simulink model "nms_sim_2D_cost"  (R2024b)
settings: Solver=ode15s  StartTime=0.0  StopTime=t_sim  MaxStep=dt_max  EnableMultiTasking=on
values from neighbouring files (symbols this model uses):
  a_BFSH = param_ctrl(35)*1    [setCtrlPar_optim_CPGreflex2001_2D.m]
  a_GAS = param_ctrl(37)*1    [setCtrlPar_optim_CPGreflex2001_2D.m]
  a_GLU = param_ctrl(31)*1    [setCtrlPar_optim_CPGreflex2001_2D.m]
  a_HAM = param_ctrl(33)*1    [setCtrlPar_optim_CPGreflex2001_2D.m]
  a_HFL = param_ctrl(32)*1    [setCtrlPar_optim_CPGreflex2001_2D.m]
  a_RF = param_ctrl(34)*1    [setCtrlPar_optim_CPGreflex2001_2D.m]
  a_SOL = param_ctrl(38)*1    [setCtrlPar_optim_CPGreflex2001_2D.m]
  a_TA = param_ctrl(39)*1    [setCtrlPar_optim_CPGreflex2001_2D.m]
  a_VAS = param_ctrl(36)*1    [setCtrlPar_optim_CPGreflex2001_2D.m]
  ai = param_ctrl(96)*2.0    [setCtrlPar_optim_CPGreflex2001_2D.m]
  b_BFSH = param_ctrl(52)*.51    [setCtrlPar_optim_CPGreflex2001_2D.m]
  b_BFSHGAS = param_ctrl(55)*.51    [setCtrlPar_optim_CPGreflex2001_2D.m]
  b_BFSHHAM = param_ctrl(54)*.51    [setCtrlPar_optim_CPGreflex2001_2D.m]
  b_BFSHVAS = param_ctrl(53)*.51    [setCtrlPar_optim_CPGreflex2001_2D.m]
  b_GAS = param_ctrl(59)*.51    [setCtrlPar_optim_CPGreflex2001_2D.m]
  b_GASBFSH = param_ctrl(60)*.51    [setCtrlPar_optim_CPGreflex2001_2D.m]
  b_GASSOL = param_ctrl(61)*.51    [setCtrlPar_optim_CPGreflex2001_2D.m]
  b_GLU = param_ctrl(40)*.51    [setCtrlPar_optim_CPGreflex2001_2D.m]
  b_GLUHAM = param_ctrl(42)*.51    [setCtrlPar_optim_CPGreflex2001_2D.m]
  b_GLUHFL = param_ctrl(41)*.51    [setCtrlPar_optim_CPGreflex2001_2D.m]
  b_HAM = param_ctrl(46)*.51    [setCtrlPar_optim_CPGreflex2001_2D.m]
  b_HAMBFSH = param_ctrl(48)*.51    [setCtrlPar_optim_CPGreflex2001_2D.m]
  b_HAMGLU = param_ctrl(47)*.51    [setCtrlPar_optim_CPGreflex2001_2D.m]
  b_HFL = param_ctrl(43)*.51    [setCtrlPar_optim_CPGreflex2001_2D.m]
  b_HFLGLU = param_ctrl(44)*.51    [setCtrlPar_optim_CPGreflex2001_2D.m]
  b_HFLRF = param_ctrl(45)*.51    [setCtrlPar_optim_CPGreflex2001_2D.m]
  b_RF = param_ctrl(49)*.51    [setCtrlPar_optim_CPGreflex2001_2D.m]
  b_RFHFL = param_ctrl(50)*.51    [setCtrlPar_optim_CPGreflex2001_2D.m]
  b_RFVAS = param_ctrl(51)*.51    [setCtrlPar_optim_CPGreflex2001_2D.m]
  b_SOL = param_ctrl(62)*.51    [setCtrlPar_optim_CPGreflex2001_2D.m]
  b_SOLGAS = param_ctrl(64)*.51    [setCtrlPar_optim_CPGreflex2001_2D.m]
  b_SOLTA = param_ctrl(63)*.51    [setCtrlPar_optim_CPGreflex2001_2D.m]
  b_TA = param_ctrl(65)*.51    [setCtrlPar_optim_CPGreflex2001_2D.m]
  b_TASOL = param_ctrl(66)*.51    [setCtrlPar_optim_CPGreflex2001_2D.m]
  b_VAS = param_ctrl(56)*.51    [setCtrlPar_optim_CPGreflex2001_2D.m]
  b_VASBFSH = param_ctrl(57)*.51    [setCtrlPar_optim_CPGreflex2001_2D.m]
  b_VASRF = param_ctrl(58)*.51    [setCtrlPar_optim_CPGreflex2001_2D.m]
  bias = param_ctrl(97)*2.5    [setCtrlPar_optim_CPGreflex2001_2D.m]
  c = 0.05    [nms_MS_2D_scaled.m]
  c_jointstop = 0.3 / (pi/180)    (= 17.1887338539)    [nms_MS_2D_scaled.m]
  D12_F = 0.16    *scaleL_JPhys    [nms_MechInit_2D_scaleSkel.m]
  D12_S = 0.2460	*sub_height    [nms_MechInit_2D_scaleSkel.m]
  D12_T = 0.2450  *sub_height    [nms_MechInit_2D_scaleSkel.m]
  D12y_F = 0.039  *sub_height    [nms_MechInit_2D_scaleSkel.m]
  D12z_HAT = 0.1    [nms_MS_2D_scaled.m]
  D13_F = 0.20    *scaleL_JPhys    [nms_MechInit_2D_scaleSkel.m]
  D1G_F = 0.14    *scaleL_JPhys    [nms_MechInit_2D_scaleSkel.m]
  D1G_HAT = 0.35  *scaleL_JPhys    [nms_MechInit_2D_scaleSkel.m]
  D1G_S = (0.3 - D12y_F/4)	*scaleL_JPhys    [nms_MechInit_2D_scaleSkel.m]
  D1G_T = (0.3 - D12y_F/4)	*scaleL_JPhys    [nms_MechInit_2D_scaleSkel.m]
  D1Gy_F = D12y_F*D1G_F/D12_F    (= 0.07)    [nms_MechInit_2D_scaleSkel.m]
  d_BFSH = param_ctrl(26)*1    [setCtrlPar_optim_CPGreflex2001_2D.m]
  d_GAS = param_ctrl(28)*1    [setCtrlPar_optim_CPGreflex2001_2D.m]
  d_GLU = param_ctrl(22)*1    [setCtrlPar_optim_CPGreflex2001_2D.m]
  d_HAM = param_ctrl(24)*1    [setCtrlPar_optim_CPGreflex2001_2D.m]
  d_HFL = param_ctrl(23)*1    [setCtrlPar_optim_CPGreflex2001_2D.m]
  d_RF = param_ctrl(25)*1    [setCtrlPar_optim_CPGreflex2001_2D.m]
  d_SOL = param_ctrl(29)*1    [setCtrlPar_optim_CPGreflex2001_2D.m]
  d_TA = param_ctrl(30)*1    [setCtrlPar_optim_CPGreflex2001_2D.m]
  d_VAS = param_ctrl(27)*1    [setCtrlPar_optim_CPGreflex2001_2D.m]
  DeltaThRef = 5e-3    (= 0.005)    [nms_MS_2D_scaled.m]
  dloptBFSH = 3.0    (= 3)    [setCtrlPar_optim_CPGreflex2001_2D.m]
  dloptGAS = 3.0    (= 3)    [setCtrlPar_optim_CPGreflex2001_2D.m]
  dloptGLU = 3.0    (= 3)    [setCtrlPar_optim_CPGreflex2001_2D.m]
  dloptHAM = 3.0    (= 3)    [setCtrlPar_optim_CPGreflex2001_2D.m]
  dloptHFL = 3.0    (= 3)    [setCtrlPar_optim_CPGreflex2001_2D.m]
  dloptRF = 3.0    (= 3)    [setCtrlPar_optim_CPGreflex2001_2D.m]
  dloptSOL = 3.0    (= 3)    [setCtrlPar_optim_CPGreflex2001_2D.m]
  dloptTA = 3.0    (= 3)    [setCtrlPar_optim_CPGreflex2001_2D.m]
  dloptVAS = 3.0    (= 3)    [setCtrlPar_optim_CPGreflex2001_2D.m]
  ec_BFSH = param_ctrl(80)*0.15    [setCtrlPar_optim_CPGreflex2001_2D.m]
  ec_GAS = param_ctrl(82)*0.15    [setCtrlPar_optim_CPGreflex2001_2D.m]
  ec_GLU = param_ctrl(76)*0.15    [setCtrlPar_optim_CPGreflex2001_2D.m]
  ec_HAM = param_ctrl(78)*0.15    [setCtrlPar_optim_CPGreflex2001_2D.m]
  ec_HFL = param_ctrl(77)*0.15    [setCtrlPar_optim_CPGreflex2001_2D.m]
  ec_RF = param_ctrl(79)*0.15    [setCtrlPar_optim_CPGreflex2001_2D.m]
  ec_TA = param_ctrl(84)*0.15    [setCtrlPar_optim_CPGreflex2001_2D.m]
  ec_VAS = param_ctrl(81)*0.15    [setCtrlPar_optim_CPGreflex2001_2D.m]
  eref = 0.04    [nms_MS_2D_scaled.m]
  eref_GAS = 0.1    [nms_MS_2D_scaled.m]
  eref_SOL = 0.1    [nms_MS_2D_scaled.m]
  es_BFSH = param_ctrl(89)*0.15    [setCtrlPar_optim_CPGreflex2001_2D.m]
  es_GAS = param_ctrl(91)*0.15    [setCtrlPar_optim_CPGreflex2001_2D.m]
  es_GLU = param_ctrl(85)*0.15    [setCtrlPar_optim_CPGreflex2001_2D.m]
  es_HAM = param_ctrl(87)*0.15    [setCtrlPar_optim_CPGreflex2001_2D.m]
  es_HFL = param_ctrl(86)*0.15    [setCtrlPar_optim_CPGreflex2001_2D.m]
  es_RF = param_ctrl(88)*0.15    [setCtrlPar_optim_CPGreflex2001_2D.m]
  es_TA = param_ctrl(93)*0.15    [setCtrlPar_optim_CPGreflex2001_2D.m]
  es_VAS = param_ctrl(90)*0.15    [setCtrlPar_optim_CPGreflex2001_2D.m]
  FmaxBFSH = 350    [nms_MS_2D_scaled.m]
  FmaxGAS = 2000    [nms_MS_2D_scaled.m]
  FmaxGLU = 4000    [nms_MS_2D_scaled.m]
  FmaxHAM = 2000    [nms_MS_2D_scaled.m]
  FmaxHFL = 2000    [nms_MS_2D_scaled.m]
  FmaxRF = 850    [nms_MS_2D_scaled.m]
  FmaxSOL = 4000    [nms_MS_2D_scaled.m]
  FmaxTA = 800    [nms_MS_2D_scaled.m]
  FmaxVAS = 5000    [nms_MS_2D_scaled.m]
  g = 9.81    [nms_MS_2D_scaled.m]
  gamma_4 = param_ctrl(11) * 1.7    [setCtrlPar_optim_CPGreflexsynergy2023_2D.m]
  h_BFSH = param_ctrl(71)*.1    [setCtrlPar_optim_CPGreflex2001_2D.m]
  h_GAS = param_ctrl(73)*.1    [setCtrlPar_optim_CPGreflex2001_2D.m]
  h_GLU = param_ctrl(67)*.1    [setCtrlPar_optim_CPGreflex2001_2D.m]
  h_HAM = param_ctrl(69)*.1    [setCtrlPar_optim_CPGreflex2001_2D.m]
  h_HFL = param_ctrl(68)*.1    [setCtrlPar_optim_CPGreflex2001_2D.m]
  h_RF = param_ctrl(70)*.1    [setCtrlPar_optim_CPGreflex2001_2D.m]
  h_SOL = param_ctrl(74)*.1    [setCtrlPar_optim_CPGreflex2001_2D.m]
  h_TA = param_ctrl(75)*.1    [setCtrlPar_optim_CPGreflex2001_2D.m]
  h_VAS = param_ctrl(72)*.1    [setCtrlPar_optim_CPGreflex2001_2D.m]
  HLCtrlPar = [theta_tgt l_clr alpha_tgt alpha_cd alpha_cv]    [setCtrlPar_optim_reflex2015_2D.m]
  In_F = 0.005    *scaleM*scaleL_JPhys^2    [nms_MechInit_2D_scaleSkel.m]
  In_HAT = 2.5    *scaleM*scaleL_JPhys^2    [nms_MechInit_2D_scaleSkel.m]
  In_S = 0.05     *scaleM*scaleL_JPhys^2    [nms_MechInit_2D_scaleSkel.m]
  In_T = 0.15     *scaleM*scaleL_JPhys^2    [nms_MechInit_2D_scaleSkel.m]
  init_exc = 0.01    [setInitPar_optim_2D.m]
  init_fm = 0.01    [setInitPar_optim_2D.m]
  init_lce = 1    [setInitPar_optim_2D.m]
  init_LCPG = param_ctrl(12) * 0.01    [setCtrlPar_optim_CPGreflexsynergy2023_2D.m]
  init_LStance = 1    [setInitPar_optim_2D.m]
  init_N1 = osc_signal1(phi_off_osc_ind)    [setCtrlPar_optim_CPGreflex2001_2D.m]
  ... (+441 more)
undefined symbols (not defined in the file or in its folder): cost_act_exponent, cost_v_tgt, flag_controller, Newton, nStep_obj, nStep_startKin, Raphson, sgn, SSW_kin, terrain_slope_angle, v_plateS1, X, Y, Z
libraries: nesl_utility x94, sm_lib x90, simulink x28, simulink_extras x12
(part 19 of 20)

== system nms_sim_2D_cost/Reflex Controller/Lower Control Layer (Spinal Cord)/R Swing Phase ==
  note: Left Swing Phase Control
  note: 0: Pre-excitations
  note: M6: swing hip
  note: M7: flex knee
  note: M8: hold knee
  note: M9: stop leg
  note: M10: prepare stance
  note: M5: flex ankle
  CtrlPar : Inport
  Stance : Inport  Port=2
  a_tgt : Inport  Port=3
  l_clr : Inport  Port=4
  LceRF : Inport  Port=5
  VceRF : Inport  Port=6
  LceHAM : Inport  Port=7
  VceHAM : Inport  Port=8
  lceBFSH : Inport  Port=9
  VceVAS : Inport  Port=10
  VceBFSH : Inport  Port=11
  LceHFL : Inport  Port=12
  LceGLU : Inport  Port=13
  LceVAS : Inport  Port=14
  LceTA : Inport  Port=15
  Enable : EnablePort  StatesWhenEnabling=reset  ZeroCross=off
  Constant1 : Constant  Value=0  OutDataTypeStr=boolean
  Constant10 : Constant  Value=leg_l
  Constant2 : Constant
  Constant3 : Constant
  Constant5 : Constant
  Demux1 : Demux  Outputs=2
  Demux2 : Demux  Outputs=2
  Demux4 : Demux  Outputs=9
  Divide{1..8,22} (9 alike) : Product
  Gain1 : Gain  Gain=-1
  Logical Operator : Logic  Operator=NOT  AllPortsSameDT=off  OutDataTypeStr=boolean
  Logical Operator1 : Logic  AllPortsSameDT=off  OutDataTypeStr=boolean
  Logical Operator2 : Logic  Operator=NOT  AllPortsSameDT=off  OutDataTypeStr=boolean
  Mux1 : Mux  Inputs=3
  Mux2 : Mux  Inputs=2
  Mux3 : Mux  Inputs=2
  Mux4 : Mux  Inputs=3
  Mux8 : Mux  Inputs=2
  Relational Operator : RelationalOperator  Operator=<=  OutDataTypeStr=boolean  ZeroCross=off  InputSameDT=off
  S-R Flip-Flop : simulink_extras/Flip Flops/S-R Flip-Flop  initial_condition=0
  Sum1 : Sum  Inputs=-+|  InputSameDT=on  SaturateOnIntegerOverflow=on  OutDataTypeStr=Inherit: Same as first input
  Sum10 : Sum  Inputs=++|  InputSameDT=on  SaturateOnIntegerOverflow=on  OutDataTypeStr=Inherit: Same as first input
  Sum13 : Sum  Inputs=|+-  InputSameDT=on  SaturateOnIntegerOverflow=on  OutDataTypeStr=Inherit: Same as first input
  Sum14 : Sum  Inputs=|+-  InputSameDT=on  SaturateOnIntegerOverflow=on  OutDataTypeStr=Inherit: Same as first input
  Sum2 : Sum  Inputs=++|  InputSameDT=on  SaturateOnIntegerOverflow=on  OutDataTypeStr=Inherit: Same as first input
  Sum3 : Sum  Inputs=-+|  InputSameDT=on  SaturateOnIntegerOverflow=on  OutDataTypeStr=Inherit: Same as first input
  Sum4 : Sum  Inputs=|+-  InputSameDT=on  SaturateOnIntegerOverflow=on  OutDataTypeStr=Inherit: Same as first input
  Sum5 : Sum  Inputs=+-|  InputSameDT=on  SaturateOnIntegerOverflow=on  OutDataTypeStr=Inherit: Same as first input
  Sum6 : Sum  Inputs=|++  InputSameDT=on  SaturateOnIntegerOverflow=on  OutDataTypeStr=Inherit: Same as first input
  Sum7 : Sum  Inputs=|++  InputSameDT=on  SaturateOnIntegerOverflow=on  OutDataTypeStr=Inherit: Same as first input
  Sum8 : Sum  Inputs=++|  InputSameDT=on  SaturateOnIntegerOverflow=on  OutDataTypeStr=Inherit: Same as first input
  Sum9 : Sum  Inputs=+-|  InputSameDT=on  SaturateOnIntegerOverflow=on  OutDataTypeStr=Inherit: Same as first input
  Terminator : Terminator
  kneei_flexion from alpha : Subsystem  TreatAsAtomicUnit=on
  kneeii_damp and hold & kneeiii_leg stop & kneeiv_stance preparation : Subsystem  TreatAsAtomicUnit=on
  negative half : Saturate  UpperLimit=0  LowerLimit=-inf  ZeroCross=off
  negative half1 : Saturate  UpperLimit=0  LowerLimit=-inf  ZeroCross=off
  negative half2 : Saturate  UpperLimit=0  LowerLimit=-inf  ZeroCross=off
  parSwA : Selector  InputPortWidth=Sw_i  IndexOptions=Index vector (dialog)  Indices=parSwA_i  OutputSizes=1
  parSwH : Selector  InputPortWidth=Sw_i  IndexOptions=Index vector (dialog)  Indices=parSwH_i  OutputSizes=1
  parSwKi : Selector  InputPortWidth=Sw_i  IndexOptions=Index vector (dialog)  Indices=parSwKi_i  OutputSizes=1
  parSwPhi : Selector  InputPortWidth=Sw_i  IndexOptions=Index vector (dialog)  Indices=parSwPhi_i  OutputSizes=1
  parSwPreE : Selector  InputPortWidth=Sw_i  IndexOptions=Index vector (dialog)  Indices=parSwPreE_i  OutputSizes=1
  phi_clr : Fcn  Expr=acos((u(2)^2+u(3)^2-u(1)^2)/(2*u(2)*u(3)))
  positive half1 : Saturate  UpperLimit=inf  LowerLimit=0  ZeroCross=off
  positive half2 : Saturate  UpperLimit=inf  LowerLimit=0  ZeroCross=off
  positive half3 : Saturate  UpperLimit=inf  LowerLimit=0  ZeroCross=off
  E_Sw_0 : Outport  OutputWhenDisabled=reset  InitialOutput=0  VectorParamsAs1DForOutWhenUnconnected=off
  E_M5_Sw [TA] : Outport  Port=2  OutputWhenDisabled=reset  InitialOutput=0  VectorParamsAs1DForOutWhenUnconnected=off
  E_M6 [HFL GLU] : Outport  Port=3  OutputWhenDisabled=reset  InitialOutput=0  VectorParamsAs1DForOutWhenUnconnected=off
  E_M7_DS [BFSH] : Outport  Port=4  OutputWhenDisabled=reset  InitialOutput=0  VectorParamsAs1DForOutWhenUnconnected=off
  E_M7_Sw [BFSH] : Outport  Port=5  OutputWhenDisabled=reset  InitialOutput=0  VectorParamsAs1DForOutWhenUnconnected=off
  M8 [RF BFSH] : Outport  Port=6  OutputWhenDisabled=reset  InitialOutput=0  VectorParamsAs1DForOutWhenUnconnected=off
  M9 [HAM BFSH GAS] : Outport  Port=7  OutputWhenDisabled=reset  InitialOutput=0  VectorParamsAs1DForOutWhenUnconnected=off
  M10 [HFL GLU VAS] : Outport  Port=8  OutputWhenDisabled=reset  InitialOutput=0  VectorParamsAs1DForOutWhenUnconnected=off
  wires:
  CtrlPar/1 -> parSwA/1, parSwPreE/1, parSwH/1, kneeii_damp and hold & kneeiii_leg stop & kneeiv_stance preparation/1(CtrlPar), parSwPhi/1, parSwKi/1
  parSwH/1 -> Demux4/1
  Constant5/1 -> Sum10/1
  a_tgt/1 -> Sum2/1, kneeii_damp and hold & kneeiii_leg stop & kneeiv_stance preparation/2(a_tgt), Sum13/1
  Demux4/2 -> Sum13/2  "aRef_RF"
  Sum13/1 -> Divide22/2
  Demux4/1 -> Divide22/1  "a2lopt_RF"
  Divide22/1 -> Sum10/2
  Sum10/1 -> Sum1/1  "lceOffRF"
  Sum1/1 -> positive half2/1  "del_LceRF"
  positive half2/1 -> Divide5/1  "del_lce"
  Demux4/3 -> Divide5/2  "LGainRF_HFL"
  Demux4/6 -> Sum2/2  "a_del"
  Sum2/1 -> Sum4/1  "a_thr"
  Demux4/7 -> Sum4/2  "aRef_HAM"
  Sum4/1 -> Divide1/2
  Demux4/5 -> Divide1/1  "a2lopt_HAM"
  Constant2/1 -> Sum5/1
  Divide1/1 -> Sum5/2
  Sum3/1 -> positive half1/1
  positive half1/1 -> Divide2/1
  Demux4/8 -> Divide2/2  "LGainHAM_GLU"
  Sum5/1 -> Sum3/1  "lceOffHAM"
  LceHAM/1 -> Sum3/2, kneeii_damp and hold & kneeiii_leg stop & kneeiv_stance preparation/4(LceHAM)
  Gain1/1 -> Divide3/1
  negative half/1 -> Gain1/1  "-VceRF"
  parSwKi/1 -> Divide3/2  "VGainRF_BFSH"
  Divide3/1 -> kneei_flexion from alpha/1(SBFSH), E_M7_DS [BFSH]/1  "BFSH"
  Constant1/1 -> S-R Flip-Flop/2
  S-R Flip-Flop/2 -> Terminator/1
  S-R Flip-Flop/1 -> Logical Operator/1, kneeii_damp and hold & kneeiii_leg stop & kneeiv_stance preparation/Enable
  Logical Operator/1 -> kneei_flexion from alpha/Enable
  lceBFSH/1 -> Relational Operator/1
  Mux8/1 -> phi_clr/1
  l_clr/1 -> Mux8/1
  Constant10/1 -> Mux8/2
  parSwPhi/1 -> Demux1/1
  Sum9/1 -> Divide4/2
  Demux1/1 -> Divide4/1  "phi2lopt_BFSH"
  Demux1/2 -> Sum9/2  "phiRef_BFSH"
  phi_clr/1 -> Sum9/1
  Constant3/1 -> Sum8/1
  Divide4/1 -> Sum8/2
  Sum8/1 -> Relational Operator/2  "lceOffLClr_BFSH"
  VceBFSH/1 -> kneeii_damp and hold & kneeiii_leg stop & kneeiv_stance preparation/7(VceBFSH)
  LceHFL/1 -> kneeii_damp and hold & kneeiii_leg stop & kneeiv_stance preparation/9(LceHFL)  "LceHFL"
  LceGLU/1 -> kneeii_damp and hold & kneeiii_leg stop & kneeiv_stance preparation/10(LceGLU)
  LceVAS/1 -> kneeii_damp and hold & kneeiii_leg stop & kneeiv_stance preparation/11(LceVAS)
  kneeii_damp and hold & kneeiii_leg stop & kneeiv_stance preparation/6(SHFL_Sw_kiv) -> Mux1/1
  kneeii_damp and hold & kneeiii_leg stop & kneeiv_stance preparation/7(SGLU_Sw_kiv) -> Mux1/2
  kneei_flexion from alpha/1(SBFSH_Sw_ki) -> E_M7_Sw [BFSH]/1
  kneeii_damp and hold & kneeiii_leg stop & kneeiv_stance preparation/2(SBFSH_Sw_kii) -> Mux3/2
  kneeii_damp and hold & kneeiii_leg stop & kneeiv_stance preparation/4(SBFSH_Sw_kiii) -> Mux4/2
  parSwA/1 -> Demux2/1
  Demux2/1 -> Divide6/1  "LGainTA"
  Sum14/1 -> positive half3/1
  LceTA/1 -> Sum14/1
  positive half3/1 -> Divide6/2
  Demux2/2 -> Sum14/2  "LceOffTA"
  Logical Operator1/1 -> S-R Flip-Flop/1
  Relational Operator/1 -> Logical Operator1/2
  Stance/1 -> Logical Operator2/1
  Logical Operator2/1 -> Logical Operator1/1
  parSwPreE/1 -> E_Sw_0/1
  kneeii_damp and hold & kneeiii_leg stop & kneeiv_stance preparation/3(SHAM_Sw_kiii) -> Mux4/1  "HAM"
  kneeii_damp and hold & kneeiii_leg stop & kneeiv_stance preparation/1(SRF_Sw_kii) -> Mux3/1  "RF"
  kneeii_damp and hold & kneeiii_leg stop & kneeiv_stance preparation/8(SVAS_Sw_kiv) -> Mux1/3  "VAS"
  Divide6/1 -> E_M5_Sw [TA]/1  "TA"
  kneeii_damp and hold & kneeiii_leg stop & kneeiv_stance preparation/5(SGAS_Sw_kiii) -> Mux4/3  "GAS"
  Mux2/1 -> E_M6 [HFL GLU]/1
  Mux3/1 -> M8 [RF BFSH]/1
  Mux4/1 -> M9 [HAM BFSH GAS]/1
  Mux1/1 -> M10 [HFL GLU VAS]/1
  LceRF/1 -> Sum1/2, kneeii_damp and hold & kneeiii_leg stop & kneeiv_stance preparation/3(LceRF)  "LceRF"
  VceVAS/1 -> kneeii_damp and hold & kneeiii_leg stop & kneeiv_stance preparation/6(VceVAS)
  Demux4/4 -> Divide7/1  "Sw_VGainRF_HFL"
  Demux4/9 -> Divide8/1  "Sw_VGainHAM_GLU"
  VceRF/1 -> negative half1/1, kneeii_damp and hold & kneeiii_leg stop & kneeiv_stance preparation/8(VceRF), negative half/1  "VceRF"
  VceHAM/1 -> kneeii_damp and hold & kneeiii_leg stop & kneeiv_stance preparation/5(VceHAM), negative half2/1
  Divide5/1 -> Sum6/1  "HFL"
  Divide7/1 -> Sum6/2
  Sum6/1 -> Mux2/1  "HFL"
  negative half1/1 -> Divide7/2
  negative half2/1 -> Divide8/2
  Divide2/1 -> Sum7/1  "GLU"
  Sum7/1 -> Mux2/2  "GLU"
  Divide8/1 -> Sum7/2

== system nms_sim_2D_cost/Body Mechanics/LBall Contact/2D Contact/Friction Switch ==
  note: Static/Kinetic Friction Switch
  Slide! : Inport
  Stick! : Inport  Port=2
  Memory : Memory
  S-R Flip-Flop : simulink_extras/Flip Flops/S-R Flip-Flop  initial_condition=0
  Terminator : Terminator
  Stiction : Outport  VectorParamsAs1DForOutWhenUnconnected=off
  wires:
  S-R Flip-Flop/1 -> Memory/1
  S-R Flip-Flop/2 -> Terminator/1
  Stick!/1 -> S-R Flip-Flop/1
  Slide!/1 -> S-R Flip-Flop/2
  Memory/1 -> Stiction/1

== system nms_sim_2D_cost/Body Mechanics/LBall Contact/2D Contact/Kinetic Friction Model ==
  note: Kinetic Friction Model
  note: Footpoint Determiner
  note: Sliding Limit Detector
  note: Normal Ground Friction
  note: Tangential Ground Friction
  vel [m/s m/s] : Inport
  pos [m m] : Inport  Port=2
  RefPt [m m] : Inport  Port=3
  nVec [m m] : Inport  Port=4
  Enable : EnablePort  StatesWhenEnabling=reset  ZeroCross=off
  Constant : Constant  Value=vLimit
  Constant1 : Constant  Value=[0 0 1]'
  FixPt Relational Operator : RelationalOperator  Operator=>  OutDataTypeStr=boolean  ZeroCross=off  InputSameDT=off
  Gain3 : Gain  Gain=k_gn
  Gain4 : Gain  Gain=1/v_gn_max
  Memory : Memory
  Mux1 : Mux  Inputs=2
  Mux2 : Mux  Inputs=2
  Negative : simulink/Logic and Bit Operations/Compare To Zero  relop=<  OutDataTypeStr=boolean
  Normal Axis Ground Force : Fcn  Expr="u(1)  *  (1-u(2)) * (u(2)<1)"
  Product : Product  RndMeth=Zero
  Product1 : Product  RndMeth=Zero
  Selector1 : Selector  InputPortWidth=3  IndexOptions=Index vector (dialog)  Indices=3  OutputSizes=1
  Selector2 : Selector  InputPortWidth=3  IndexOptions=Index vector (dialog)  Indices=[1 2]  OutputSizes=1
  Sum : Sum  Inputs=|+-
  Switch : Switch  Criteria=u2 > Threshold  Threshold=0.9*vLimit  SaturateOnIntegerOverflow=off  InputSameDT=off
      settings: AttributesFormatString=>%<Threshold>?
  Vector Norm : Subsystem
  d_n : DotProduct  OutDataTypeStr=Inherit: Inherit via internal rule
  qnVec : Sum  Inputs=-+
  reverse direction : Gain  Gain=-1
  sliding friction coefficient : Gain  Gain=mu_slide
  tVec : Product  Inputs=*/  RndMeth=Zero
  v_n : DotProduct  OutDataTypeStr=Inherit: Inherit via internal rule
  v_nVec : Product  RndMeth=Zero
  v_tVec : Sum  Inputs=-+|
  RefPtFP [m m] : Outport  InitialOutput=[0 0]  VectorParamsAs1DForOutWhenUnconnected=off
      settings: AttributesFormatString=initial = '%<InitialOutput>'\nwhen disabled = '%<OutputWhenDisabled>'
  posFP [m m] : Outport  Port=2  InitialOutput=[0 0]  VectorParamsAs1DForOutWhenUnconnected=off
      settings: AttributesFormatString=initial = '%<InitialOutput>'\nwhen disabled = '%<OutputWhenDisabled>'
  nVec FP [m m] : Outport  Port=3  InitialOutput=0  VectorParamsAs1DForOutWhenUnconnected=off
      settings: AttributesFormatString=initial = '%<InitialOutput>'\nwhen disabled = '%<OutputWhenDisabled>'
  Stiction! : Outport  Port=4  OutputWhenDisabled=reset  InitialOutput=0  VectorParamsAs1DForOutWhenUnconnected=off
      settings: AttributesFormatString=initial = '%<InitialOutput>'\nwhen disabled = '%<OutputWhenDisabled>'
  F_t Slide [N N] : Outport  Port=5  OutputWhenDisabled=reset  InitialOutput=[0 0]  VectorParamsAs1DForOutWhenUnconnected=off
      settings: AttributesFormatString=initial = '%<InitialOutput>'\nwhen disabled = '%<OutputWhenDisabled>'
  F_n Slide [N N] : Outport  Port=6  OutputWhenDisabled=reset  InitialOutput=[0 0]  VectorParamsAs1DForOutWhenUnconnected=off
      settings: AttributesFormatString=initial = '%<InitialOutput>'\nwhen disabled = '%<OutputWhenDisabled>'
  wires:
  Normal Axis Ground Force/1 -> sliding friction coefficient/1, Product1/2
  Product/1 -> F_t Slide [N N]/1
  FixPt Relational Operator/1 -> Stiction!/1
  Memory/1 -> FixPt Relational Operator/2
  Negative/1 -> FixPt Relational Operator/1, Memory/1
  Vector Norm/1(norm) -> Sum/1, Switch/2, Mux2/2
  Sum/1 -> Negative/1
  Constant/1 -> Sum/2
  Mux1/1 -> Normal Axis Ground Force/1
  Gain3/1 -> Mux1/1
  Gain4/1 -> Mux1/2
  nVec [m m]/1 -> v_n/1, v_nVec/2, d_n/2, Product1/1, nVec FP [m m]/1
  d_n/1 -> Gain3/1
  vel [m/s m/s]/1 -> v_n/2, v_tVec/2
  v_n/1 -> Gain4/1, v_nVec/1
  v_nVec/1 -> v_tVec/1
  v_tVec/1 -> Vector Norm/1(vec), Mux2/1
  sliding friction coefficient/1 -> Product/1
  reverse direction/1 -> Product/2
  Product1/1 -> F_n Slide [N N]/1
  tVec/1 -> reverse direction/1
  Constant1/1 -> Switch/3
  Mux2/1 -> Switch/1
  Selector1/1 -> tVec/2
  Selector2/1 -> tVec/1
  pos [m m]/1 -> posFP [m m]/1, qnVec/1
  qnVec/1 -> d_n/1
  RefPt [m m]/1 -> qnVec/2, RefPtFP [m m]/1
  Switch/1 -> Selector2/1, Selector1/1

== system nms_sim_2D_cost/Body Mechanics/LBall Contact/2D Contact/Static Friction Model ==
  note: Stiction Limit Detector
  note: Static Friction Model
  note: Zero multiplication prevents
      | horizontal friction model from
      | oscillating between static and kinetic
      | friction when the vertical force is zero but
      | the ground level is not yet reached
      | in the upward motion
  note: (distance to
      | surface)
  note: Tangential Ground Reaction Force
  pos [m] : Inport
  vel [m/s m/s] : Inport  Port=2
  RefPtFP [m m] : Inport  Port=3
  posFP [m] : Inport  Port=4
  nVecFP [m m] : Inport  Port=5
  Enable : EnablePort  StatesWhenEnabling=reset  ZeroCross=off
  Abs : Abs  SaturateOnIntegerOverflow=off
  Check Vertical Friction : Product  RndMeth=Zero
  Constant : Constant
  Dpos_n : DotProduct  OutDataTypeStr=Inherit: Inherit via internal rule
  Dpos_nVec : Product  RndMeth=Zero
  Dpos_tVec : Sum  Inputs=|+-
  FixPt Relational Operator : RelationalOperator  Operator=>  OutDataTypeStr=boolean  ZeroCross=off  InputSameDT=off
  Gain : Gain  Gain=-1
  Gain1 : Gain  Gain=k_gn
  Gain2 : Gain  Gain=1/v_gn_max
  Gain3 : Gain  Gain=k_gt
  Gain5 : Gain  Gain=1/v_gt_max
  Memory : Memory
  Mux2 : Mux  Inputs=2
  Normal Ground Reaction Force : Fcn  Expr="u(1)  *  (1-u(2)) * (u(2)<1)"
  Positive : simulink/Logic and Bit Operations/Compare To Zero  relop=>  OutDataTypeStr=boolean
  Positive1 : simulink/Logic and Bit Operations/Compare To Zero  relop=>  OutDataTypeStr=boolean
  Product1 : Product  RndMeth=Zero
  Sign : Signum  ZeroCross=off
  Sum : Sum  Inputs=-+
  Sum1 : Sum  Inputs=|+-
  Sum2 : Sum  Inputs=|+-
  Vector Norm : Subsystem
  d_n : DotProduct  OutDataTypeStr=Inherit: Inherit via internal rule
  stiction limit force : Gain  Gain=mu_stick
  sum : Sum  Inputs=++|
  tVec1 : Product  Inputs=**  RndMeth=Zero
  tVec2 : Product  Inputs=**  RndMeth=Zero
  v_n : DotProduct  OutDataTypeStr=Inherit: Inherit via internal rule
  v_nVec : Product  RndMeth=Zero
  v_tVec : Sum  Inputs=-+|
  F_n Stick [N N] : Outport  OutputWhenDisabled=reset  InitialOutput=[0 0]  VectorParamsAs1DForOutWhenUnconnected=off
      settings: AttributesFormatString=initial = '%<InitialOutput>'\nwhen disabled = '%<OutputWhenDisabled>'
  F_t Stick [N N] : Outport  Port=2  OutputWhenDisabled=reset  InitialOutput=[0 0]  VectorParamsAs1DForOutWhenUnconnected=off
      settings: AttributesFormatString=when disabled: %<OutputWhenDisabled>\ninitial: %<InitialOutput>
  Sliding! : Outport  Port=3  OutputWhenDisabled=reset  InitialOutput=0  VectorParamsAs1DForOutWhenUnconnected=off
      settings: AttributesFormatString=when disabled: %<OutputWhenDisabled>\ninitial: %<InitialOutput>
  wires:
  Sum/1 -> Positive/1
  Memory/1 -> FixPt Relational Operator/2
  Positive/1 -> FixPt Relational Operator/1, Memory/1
  FixPt Relational Operator/1 -> Sliding!/1
  Abs/1 -> Sum/1
  stiction limit force/1 -> Abs/1
  Positive1/1 -> Check Vertical Friction/2
  Check Vertical Friction/1 -> Vector Norm/1(vec), F_t Stick [N N]/1
  Normal Ground Reaction Force/1 -> Product1/2, stiction limit force/1, Positive1/1
  Mux2/1 -> Normal Ground Reaction Force/1
  Gain1/1 -> Mux2/1
  Gain2/1 -> Mux2/2
  nVecFP [m m]/1 -> d_n/1, v_n/2, Dpos_n/1, Dpos_nVec/1, v_nVec/2, Product1/1
  d_n/1 -> Gain1/1
  vel [m/s m/s]/1 -> v_tVec/2, v_n/1
  v_n/1 -> v_nVec/1, Gain2/1
  v_nVec/1 -> v_tVec/1
  v_tVec/1 -> Gain5/1
  Product1/1 -> F_n Stick [N N]/1
  pos [m]/1 -> Sum2/1, Sum1/2
  posFP [m]/1 -> Sum2/2
  Sum2/1 -> Dpos_n/2, Dpos_tVec/1  "Dpos"
  Dpos_n/1 -> Dpos_nVec/2
  Dpos_nVec/1 -> Dpos_tVec/2
  Dpos_tVec/1 -> Gain3/1
  Gain3/1 -> Sign/1, tVec2/2
  Sign/1 -> tVec1/2
  tVec1/1 -> sum/2
  Constant/1 -> sum/1
  sum/1 -> tVec2/1
  tVec2/1 -> Gain/1
  Gain/1 -> Check Vertical Friction/1
  Vector Norm/1(norm) -> Sum/2
  RefPtFP [m m]/1 -> Sum1/1
  Sum1/1 -> d_n/2
  Gain5/1 -> tVec1/1

== system nms_sim_2D_cost/Body Mechanics/LHeel Contact/2D Contact/Friction Switch ==
  note: Static/Kinetic Friction Switch
  Slide! : Inport
  Stick! : Inport  Port=2
  Memory : Memory
  S-R Flip-Flop : simulink_extras/Flip Flops/S-R Flip-Flop  initial_condition=0
  Terminator : Terminator
  Stiction : Outport  VectorParamsAs1DForOutWhenUnconnected=off
  wires:
  S-R Flip-Flop/1 -> Memory/1
  S-R Flip-Flop/2 -> Terminator/1
  Stick!/1 -> S-R Flip-Flop/1
  Slide!/1 -> S-R Flip-Flop/2
  Memory/1 -> Stiction/1

== system nms_sim_2D_cost/Body Mechanics/LHeel Contact/2D Contact/Kinetic Friction Model ==
  note: Kinetic Friction Model
  note: Footpoint Determiner
  note: Sliding Limit Detector
  note: Normal Ground Friction
  note: Tangential Ground Friction
  vel [m/s m/s] : Inport
  pos [m m] : Inport  Port=2
  RefPt [m m] : Inport  Port=3
  nVec [m m] : Inport  Port=4
  Enable : EnablePort  StatesWhenEnabling=reset  ZeroCross=off
  Constant : Constant  Value=vLimit
  Constant1 : Constant  Value=[0 0 1]'
  FixPt Relational Operator : RelationalOperator  Operator=>  OutDataTypeStr=boolean  ZeroCross=off  InputSameDT=off
  Gain3 : Gain  Gain=k_gn
  Gain4 : Gain  Gain=1/v_gn_max
  Memory : Memory
  Mux1 : Mux  Inputs=2
  Mux2 : Mux  Inputs=2
  Negative : simulink/Logic and Bit Operations/Compare To Zero  relop=<  OutDataTypeStr=boolean
  Normal Axis Ground Force : Fcn  Expr="u(1)  *  (1-u(2)) * (u(2)<1)"
  Product : Product  RndMeth=Zero
  Product1 : Product  RndMeth=Zero
  Selector1 : Selector  InputPortWidth=3  IndexOptions=Index vector (dialog)  Indices=3  OutputSizes=1
  Selector2 : Selector  InputPortWidth=3  IndexOptions=Index vector (dialog)  Indices=[1 2]  OutputSizes=1
  Sum : Sum  Inputs=|+-
  Switch : Switch  Criteria=u2 > Threshold  Threshold=0.9*vLimit  SaturateOnIntegerOverflow=off  InputSameDT=off
      settings: AttributesFormatString=>%<Threshold>?
  Vector Norm : Subsystem
  d_n : DotProduct  OutDataTypeStr=Inherit: Inherit via internal rule
  qnVec : Sum  Inputs=-+
  reverse direction : Gain  Gain=-1
  sliding friction coefficient : Gain  Gain=mu_slide
  tVec : Product  Inputs=*/  RndMeth=Zero
  v_n : DotProduct  OutDataTypeStr=Inherit: Inherit via internal rule
  v_nVec : Product  RndMeth=Zero
  v_tVec : Sum  Inputs=-+|
  RefPtFP [m m] : Outport  InitialOutput=[0 0]  VectorParamsAs1DForOutWhenUnconnected=off
      settings: AttributesFormatString=initial = '%<InitialOutput>'\nwhen disabled = '%<OutputWhenDisabled>'
  posFP [m m] : Outport  Port=2  InitialOutput=[0 0]  VectorParamsAs1DForOutWhenUnconnected=off
      settings: AttributesFormatString=initial = '%<InitialOutput>'\nwhen disabled = '%<OutputWhenDisabled>'
  nVec FP [m m] : Outport  Port=3  InitialOutput=0  VectorParamsAs1DForOutWhenUnconnected=off
      settings: AttributesFormatString=initial = '%<InitialOutput>'\nwhen disabled = '%<OutputWhenDisabled>'
  Stiction! : Outport  Port=4  OutputWhenDisabled=reset  InitialOutput=0  VectorParamsAs1DForOutWhenUnconnected=off
      settings: AttributesFormatString=initial = '%<InitialOutput>'\nwhen disabled = '%<OutputWhenDisabled>'
  F_t Slide [N N] : Outport  Port=5  OutputWhenDisabled=reset  InitialOutput=[0 0]  VectorParamsAs1DForOutWhenUnconnected=off
      settings: AttributesFormatString=initial = '%<InitialOutput>'\nwhen disabled = '%<OutputWhenDisabled>'
  F_n Slide [N N] : Outport  Port=6  OutputWhenDisabled=reset  InitialOutput=[0 0]  VectorParamsAs1DForOutWhenUnconnected=off
      settings: AttributesFormatString=initial = '%<InitialOutput>'\nwhen disabled = '%<OutputWhenDisabled>'
  wires:
  Normal Axis Ground Force/1 -> sliding friction coefficient/1, Product1/2
  Product/1 -> F_t Slide [N N]/1
  FixPt Relational Operator/1 -> Stiction!/1
  Memory/1 -> FixPt Relational Operator/2
  Negative/1 -> FixPt Relational Operator/1, Memory/1
  Vector Norm/1(norm) -> Sum/1, Switch/2, Mux2/2
  Sum/1 -> Negative/1
  Constant/1 -> Sum/2
  Mux1/1 -> Normal Axis Ground Force/1
  Gain3/1 -> Mux1/1
  Gain4/1 -> Mux1/2
  nVec [m m]/1 -> v_n/1, v_nVec/2, d_n/2, Product1/1, nVec FP [m m]/1
  d_n/1 -> Gain3/1
  vel [m/s m/s]/1 -> v_n/2, v_tVec/2
  v_n/1 -> Gain4/1, v_nVec/1
  v_nVec/1 -> v_tVec/1
  v_tVec/1 -> Vector Norm/1(vec), Mux2/1
  sliding friction coefficient/1 -> Product/1
  reverse direction/1 -> Product/2
  Product1/1 -> F_n Slide [N N]/1
  tVec/1 -> reverse direction/1
  Constant1/1 -> Switch/3
  Mux2/1 -> Switch/1
  Selector1/1 -> tVec/2
  Selector2/1 -> tVec/1
  pos [m m]/1 -> posFP [m m]/1, qnVec/1
  qnVec/1 -> d_n/1
  RefPt [m m]/1 -> qnVec/2, RefPtFP [m m]/1
  Switch/1 -> Selector2/1, Selector1/1

== system nms_sim_2D_cost/Body Mechanics/LHeel Contact/2D Contact/Static Friction Model ==
  note: Stiction Limit Detector
  note: Static Friction Model
  note: Zero multiplication prevents
      | horizontal friction model from
      | oscillating between static and kinetic
      | friction when the vertical force is zero but
      | the ground level is not yet reached
      | in the upward motion
  note: (distance to
      | surface)
  note: Tangential Ground Reaction Force
  pos [m] : Inport
  vel [m/s m/s] : Inport  Port=2
  RefPtFP [m m] : Inport  Port=3
  posFP [m] : Inport  Port=4
  nVecFP [m m] : Inport  Port=5
  Enable : EnablePort  StatesWhenEnabling=reset  ZeroCross=off
  Abs : Abs  SaturateOnIntegerOverflow=off
  Check Vertical Friction : Product  RndMeth=Zero
  Constant : Constant
  Dpos_n : DotProduct  OutDataTypeStr=Inherit: Inherit via internal rule
  Dpos_nVec : Product  RndMeth=Zero
  Dpos_tVec : Sum  Inputs=|+-
  FixPt Relational Operator : RelationalOperator  Operator=>  OutDataTypeStr=boolean  ZeroCross=off  InputSameDT=off
  Gain : Gain  Gain=-1
  Gain1 : Gain  Gain=k_gn
  Gain2 : Gain  Gain=1/v_gn_max
  Gain3 : Gain  Gain=k_gt
  Gain5 : Gain  Gain=1/v_gt_max
  Memory : Memory
  Mux2 : Mux  Inputs=2
  Normal Ground Reaction Force : Fcn  Expr="u(1)  *  (1-u(2)) * (u(2)<1)"
  Positive : simulink/Logic and Bit Operations/Compare To Zero  relop=>  OutDataTypeStr=boolean
  Positive1 : simulink/Logic and Bit Operations/Compare To Zero  relop=>  OutDataTypeStr=boolean
  Product1 : Product  RndMeth=Zero
  Sign : Signum  ZeroCross=off
  Sum : Sum  Inputs=-+
  Sum1 : Sum  Inputs=|+-
  Sum2 : Sum  Inputs=|+-
  Vector Norm : Subsystem
  d_n : DotProduct  OutDataTypeStr=Inherit: Inherit via internal rule
  stiction limit force : Gain  Gain=mu_stick
  sum : Sum  Inputs=++|
  tVec1 : Product  Inputs=**  RndMeth=Zero
  tVec2 : Product  Inputs=**  RndMeth=Zero
  v_n : DotProduct  OutDataTypeStr=Inherit: Inherit via internal rule
  v_nVec : Product  RndMeth=Zero
  v_tVec : Sum  Inputs=-+|
  F_n Stick [N N] : Outport  OutputWhenDisabled=reset  InitialOutput=[0 0]  VectorParamsAs1DForOutWhenUnconnected=off
      settings: AttributesFormatString=initial = '%<InitialOutput>'\nwhen disabled = '%<OutputWhenDisabled>'
  F_t Stick [N N] : Outport  Port=2  OutputWhenDisabled=reset  InitialOutput=[0 0]  VectorParamsAs1DForOutWhenUnconnected=off
      settings: AttributesFormatString=when disabled: %<OutputWhenDisabled>\ninitial: %<InitialOutput>
  Sliding! : Outport  Port=3  OutputWhenDisabled=reset  InitialOutput=0  VectorParamsAs1DForOutWhenUnconnected=off
      settings: AttributesFormatString=when disabled: %<OutputWhenDisabled>\ninitial: %<InitialOutput>
  wires:
  Sum/1 -> Positive/1
  Memory/1 -> FixPt Relational Operator/2
  Positive/1 -> FixPt Relational Operator/1, Memory/1
  FixPt Relational Operator/1 -> Sliding!/1
  Abs/1 -> Sum/1
  stiction limit force/1 -> Abs/1
  Positive1/1 -> Check Vertical Friction/2
  Check Vertical Friction/1 -> Vector Norm/1(vec), F_t Stick [N N]/1
  Normal Ground Reaction Force/1 -> Product1/2, stiction limit force/1, Positive1/1
  Mux2/1 -> Normal Ground Reaction Force/1
  Gain1/1 -> Mux2/1
  Gain2/1 -> Mux2/2
  nVecFP [m m]/1 -> d_n/1, v_n/2, Dpos_n/1, Dpos_nVec/1, v_nVec/2, Product1/1
  d_n/1 -> Gain1/1
  vel [m/s m/s]/1 -> v_tVec/2, v_n/1
  v_n/1 -> v_nVec/1, Gain2/1
  v_nVec/1 -> v_tVec/1
  v_tVec/1 -> Gain5/1
  Product1/1 -> F_n Stick [N N]/1
  pos [m]/1 -> Sum2/1, Sum1/2
  posFP [m]/1 -> Sum2/2
  Sum2/1 -> Dpos_n/2, Dpos_tVec/1  "Dpos"
  Dpos_n/1 -> Dpos_nVec/2
  Dpos_nVec/1 -> Dpos_tVec/2
  Dpos_tVec/1 -> Gain3/1
  Gain3/1 -> Sign/1, tVec2/2
  Sign/1 -> tVec1/2
  tVec1/1 -> sum/2
  Constant/1 -> sum/1
  sum/1 -> tVec2/1
  tVec2/1 -> Gain/1
  Gain/1 -> Check Vertical Friction/1
  Vector Norm/1(norm) -> Sum/2
  RefPtFP [m m]/1 -> Sum1/1
  Sum1/1 -> d_n/2
  Gain5/1 -> tVec1/1

== system nms_sim_2D_cost/Body Mechanics/RBall Contact/2D Contact/Friction Switch ==
  note: Static/Kinetic Friction Switch
  Slide! : Inport
  Stick! : Inport  Port=2
  Memory : Memory
  S-R Flip-Flop : simulink_extras/Flip Flops/S-R Flip-Flop  initial_condition=0
  Terminator : Terminator
  Stiction : Outport  VectorParamsAs1DForOutWhenUnconnected=off
  wires:
  S-R Flip-Flop/1 -> Memory/1
  S-R Flip-Flop/2 -> Terminator/1
  Stick!/1 -> S-R Flip-Flop/1
  Slide!/1 -> S-R Flip-Flop/2
  Memory/1 -> Stiction/1

== system nms_sim_2D_cost/Body Mechanics/RBall Contact/2D Contact/Kinetic Friction Model ==
  note: Kinetic Friction Model
  note: Footpoint Determiner
  note: Sliding Limit Detector
  note: Normal Ground Friction
  note: Tangential Ground Friction
  vel [m/s m/s] : Inport
  pos [m m] : Inport  Port=2
  RefPt [m m] : Inport  Port=3
  nVec [m m] : Inport  Port=4
  Enable : EnablePort  StatesWhenEnabling=reset  ZeroCross=off
  Constant : Constant  Value=vLimit
  Constant1 : Constant  Value=[0 0 1]'
  FixPt Relational Operator : RelationalOperator  Operator=>  OutDataTypeStr=boolean  ZeroCross=off  InputSameDT=off
  Gain3 : Gain  Gain=k_gn
  Gain4 : Gain  Gain=1/v_gn_max
  Memory : Memory
  Mux1 : Mux  Inputs=2
  Mux2 : Mux  Inputs=2
  Negative : simulink/Logic and Bit Operations/Compare To Zero  relop=<  OutDataTypeStr=boolean
  Normal Axis Ground Force : Fcn  Expr="u(1)  *  (1-u(2)) * (u(2)<1)"
  Product : Product  RndMeth=Zero
  Product1 : Product  RndMeth=Zero
  Selector1 : Selector  InputPortWidth=3  IndexOptions=Index vector (dialog)  Indices=3  OutputSizes=1
  Selector2 : Selector  InputPortWidth=3  IndexOptions=Index vector (dialog)  Indices=[1 2]  OutputSizes=1
  Sum : Sum  Inputs=|+-
  Switch : Switch  Criteria=u2 > Threshold  Threshold=0.9*vLimit  SaturateOnIntegerOverflow=off  InputSameDT=off
      settings: AttributesFormatString=>%<Threshold>?
  Vector Norm : Subsystem
  d_n : DotProduct  OutDataTypeStr=Inherit: Inherit via internal rule
  qnVec : Sum  Inputs=-+
  reverse direction : Gain  Gain=-1
  sliding friction coefficient : Gain  Gain=mu_slide
  tVec : Product  Inputs=*/  RndMeth=Zero
  v_n : DotProduct  OutDataTypeStr=Inherit: Inherit via internal rule
  v_nVec : Product  RndMeth=Zero
  v_tVec : Sum  Inputs=-+|
  RefPtFP [m m] : Outport  InitialOutput=[0 0]  VectorParamsAs1DForOutWhenUnconnected=off
      settings: AttributesFormatString=initial = '%<InitialOutput>'\nwhen disabled = '%<OutputWhenDisabled>'
  posFP [m m] : Outport  Port=2  InitialOutput=[0 0]  VectorParamsAs1DForOutWhenUnconnected=off
      settings: AttributesFormatString=initial = '%<InitialOutput>'\nwhen disabled = '%<OutputWhenDisabled>'
  nVec FP [m m] : Outport  Port=3  InitialOutput=0  VectorParamsAs1DForOutWhenUnconnected=off
      settings: AttributesFormatString=initial = '%<InitialOutput>'\nwhen disabled = '%<OutputWhenDisabled>'
  Stiction! : Outport  Port=4  OutputWhenDisabled=reset  InitialOutput=0  VectorParamsAs1DForOutWhenUnconnected=off
      settings: AttributesFormatString=initial = '%<InitialOutput>'\nwhen disabled = '%<OutputWhenDisabled>'
  F_t Slide [N N] : Outport  Port=5  OutputWhenDisabled=reset  InitialOutput=[0 0]  VectorParamsAs1DForOutWhenUnconnected=off
      settings: AttributesFormatString=initial = '%<InitialOutput>'\nwhen disabled = '%<OutputWhenDisabled>'
  F_n Slide [N N] : Outport  Port=6  OutputWhenDisabled=reset  InitialOutput=[0 0]  VectorParamsAs1DForOutWhenUnconnected=off
      settings: AttributesFormatString=initial = '%<InitialOutput>'\nwhen disabled = '%<OutputWhenDisabled>'
  wires:
  Normal Axis Ground Force/1 -> sliding friction coefficient/1, Product1/2
  Product/1 -> F_t Slide [N N]/1
  FixPt Relational Operator/1 -> Stiction!/1
  Memory/1 -> FixPt Relational Operator/2
  Negative/1 -> FixPt Relational Operator/1, Memory/1
  Vector Norm/1(norm) -> Sum/1, Switch/2, Mux2/2
  Sum/1 -> Negative/1
  Constant/1 -> Sum/2
  Mux1/1 -> Normal Axis Ground Force/1
  Gain3/1 -> Mux1/1
  Gain4/1 -> Mux1/2
  nVec [m m]/1 -> v_n/1, v_nVec/2, d_n/2, Product1/1, nVec FP [m m]/1
  d_n/1 -> Gain3/1
  vel [m/s m/s]/1 -> v_n/2, v_tVec/2
  v_n/1 -> Gain4/1, v_nVec/1
  v_nVec/1 -> v_tVec/1
  v_tVec/1 -> Vector Norm/1(vec), Mux2/1
  sliding friction coefficient/1 -> Product/1
  reverse direction/1 -> Product/2
  Product1/1 -> F_n Slide [N N]/1
  tVec/1 -> reverse direction/1
  Constant1/1 -> Switch/3
  Mux2/1 -> Switch/1
  Selector1/1 -> tVec/2
  Selector2/1 -> tVec/1
  pos [m m]/1 -> posFP [m m]/1, qnVec/1
  qnVec/1 -> d_n/1
  RefPt [m m]/1 -> qnVec/2, RefPtFP [m m]/1
  Switch/1 -> Selector2/1, Selector1/1

== system nms_sim_2D_cost/Body Mechanics/RBall Contact/2D Contact/Static Friction Model ==
  note: Stiction Limit Detector
  note: Static Friction Model
  note: Zero multiplication prevents
      | horizontal friction model from
      | oscillating between static and kinetic
      | friction when the vertical force is zero but
      | the ground level is not yet reached
      | in the upward motion
  note: (distance to
      | surface)
  note: Tangential Ground Reaction Force
  pos [m] : Inport
  vel [m/s m/s] : Inport  Port=2
  RefPtFP [m m] : Inport  Port=3
  posFP [m] : Inport  Port=4
  nVecFP [m m] : Inport  Port=5
  Enable : EnablePort  StatesWhenEnabling=reset  ZeroCross=off
  Abs : Abs  SaturateOnIntegerOverflow=off
  Check Vertical Friction : Product  RndMeth=Zero
  Constant : Constant
  Dpos_n : DotProduct  OutDataTypeStr=Inherit: Inherit via internal rule
  Dpos_nVec : Product  RndMeth=Zero
  Dpos_tVec : Sum  Inputs=|+-
  FixPt Relational Operator : RelationalOperator  Operator=>  OutDataTypeStr=boolean  ZeroCross=off  InputSameDT=off
  Gain : Gain  Gain=-1
  Gain1 : Gain  Gain=k_gn
  Gain2 : Gain  Gain=1/v_gn_max
  Gain3 : Gain  Gain=k_gt
  Gain5 : Gain  Gain=1/v_gt_max
  Memory : Memory
  Mux2 : Mux  Inputs=2
  Normal Ground Reaction Force : Fcn  Expr="u(1)  *  (1-u(2)) * (u(2)<1)"
  Positive : simulink/Logic and Bit Operations/Compare To Zero  relop=>  OutDataTypeStr=boolean
  Positive1 : simulink/Logic and Bit Operations/Compare To Zero  relop=>  OutDataTypeStr=boolean
  Product1 : Product  RndMeth=Zero
  Sign : Signum  ZeroCross=off
  Sum : Sum  Inputs=-+
  Sum1 : Sum  Inputs=|+-
  Sum2 : Sum  Inputs=|+-
  Vector Norm : Subsystem
  d_n : DotProduct  OutDataTypeStr=Inherit: Inherit via internal rule
  stiction limit force : Gain  Gain=mu_stick
  sum : Sum  Inputs=++|
  tVec1 : Product  Inputs=**  RndMeth=Zero
  tVec2 : Product  Inputs=**  RndMeth=Zero
  v_n : DotProduct  OutDataTypeStr=Inherit: Inherit via internal rule
  v_nVec : Product  RndMeth=Zero
  v_tVec : Sum  Inputs=-+|
  F_n Stick [N N] : Outport  OutputWhenDisabled=reset  InitialOutput=[0 0]  VectorParamsAs1DForOutWhenUnconnected=off
      settings: AttributesFormatString=initial = '%<InitialOutput>'\nwhen disabled = '%<OutputWhenDisabled>'
  F_t Stick [N N] : Outport  Port=2  OutputWhenDisabled=reset  InitialOutput=[0 0]  VectorParamsAs1DForOutWhenUnconnected=off
      settings: AttributesFormatString=when disabled: %<OutputWhenDisabled>\ninitial: %<InitialOutput>
  Sliding! : Outport  Port=3  OutputWhenDisabled=reset  InitialOutput=0  VectorParamsAs1DForOutWhenUnconnected=off
      settings: AttributesFormatString=when disabled: %<OutputWhenDisabled>\ninitial: %<InitialOutput>
  wires:
  Sum/1 -> Positive/1
  Memory/1 -> FixPt Relational Operator/2
  Positive/1 -> FixPt Relational Operator/1, Memory/1
  FixPt Relational Operator/1 -> Sliding!/1
  Abs/1 -> Sum/1
  stiction limit force/1 -> Abs/1
  Positive1/1 -> Check Vertical Friction/2
  Check Vertical Friction/1 -> Vector Norm/1(vec), F_t Stick [N N]/1
  Normal Ground Reaction Force/1 -> Product1/2, stiction limit force/1, Positive1/1
  Mux2/1 -> Normal Ground Reaction Force/1
  Gain1/1 -> Mux2/1
  Gain2/1 -> Mux2/2
  nVecFP [m m]/1 -> d_n/1, v_n/2, Dpos_n/1, Dpos_nVec/1, v_nVec/2, Product1/1
  d_n/1 -> Gain1/1
  vel [m/s m/s]/1 -> v_tVec/2, v_n/1
  v_n/1 -> v_nVec/1, Gain2/1
  v_nVec/1 -> v_tVec/1
  v_tVec/1 -> Gain5/1
  Product1/1 -> F_n Stick [N N]/1
  pos [m]/1 -> Sum2/1, Sum1/2
  posFP [m]/1 -> Sum2/2
  Sum2/1 -> Dpos_n/2, Dpos_tVec/1  "Dpos"
  Dpos_n/1 -> Dpos_nVec/2
  Dpos_nVec/1 -> Dpos_tVec/2
  Dpos_tVec/1 -> Gain3/1
  Gain3/1 -> Sign/1, tVec2/2
  Sign/1 -> tVec1/2
  tVec1/1 -> sum/2
  Constant/1 -> sum/1
  sum/1 -> tVec2/1
  tVec2/1 -> Gain/1
  Gain/1 -> Check Vertical Friction/1
  Vector Norm/1(norm) -> Sum/2
  RefPtFP [m m]/1 -> Sum1/1
  Sum1/1 -> d_n/2
  Gain5/1 -> tVec1/1

== system nms_sim_2D_cost/Body Mechanics/RHeel Contact/2D Contact/Friction Switch ==
  note: Static/Kinetic Friction Switch
  Slide! : Inport
  Stick! : Inport  Port=2
  Memory : Memory
  S-R Flip-Flop : simulink_extras/Flip Flops/S-R Flip-Flop  initial_condition=0
  Terminator : Terminator
  Stiction : Outport  VectorParamsAs1DForOutWhenUnconnected=off
  wires:
  S-R Flip-Flop/1 -> Memory/1
  S-R Flip-Flop/2 -> Terminator/1
  Stick!/1 -> S-R Flip-Flop/1
  Slide!/1 -> S-R Flip-Flop/2
  Memory/1 -> Stiction/1

== system nms_sim_2D_cost/Body Mechanics/RHeel Contact/2D Contact/Kinetic Friction Model ==
  note: Kinetic Friction Model
  note: Footpoint Determiner
  note: Sliding Limit Detector
  note: Normal Ground Friction
  note: Tangential Ground Friction
  vel [m/s m/s] : Inport
  pos [m m] : Inport  Port=2
  RefPt [m m] : Inport  Port=3
  nVec [m m] : Inport  Port=4
  Enable : EnablePort  StatesWhenEnabling=reset  ZeroCross=off
  Constant : Constant  Value=vLimit
  Constant1 : Constant  Value=[0 0 1]'
  FixPt Relational Operator : RelationalOperator  Operator=>  OutDataTypeStr=boolean  ZeroCross=off  InputSameDT=off
  Gain3 : Gain  Gain=k_gn
  Gain4 : Gain  Gain=1/v_gn_max
  Memory : Memory
  Mux1 : Mux  Inputs=2
  Mux2 : Mux  Inputs=2
  Negative : simulink/Logic and Bit Operations/Compare To Zero  relop=<  OutDataTypeStr=boolean
  Normal Axis Ground Force : Fcn  Expr="u(1)  *  (1-u(2)) * (u(2)<1)"
  Product : Product  RndMeth=Zero
  Product1 : Product  RndMeth=Zero
  Selector1 : Selector  InputPortWidth=3  IndexOptions=Index vector (dialog)  Indices=3  OutputSizes=1
  Selector2 : Selector  InputPortWidth=3  IndexOptions=Index vector (dialog)  Indices=[1 2]  OutputSizes=1
  Sum : Sum  Inputs=|+-
  Switch : Switch  Criteria=u2 > Threshold  Threshold=0.9*vLimit  SaturateOnIntegerOverflow=off  InputSameDT=off
      settings: AttributesFormatString=>%<Threshold>?
  Vector Norm : Subsystem
  d_n : DotProduct  OutDataTypeStr=Inherit: Inherit via internal rule
  qnVec : Sum  Inputs=-+
  reverse direction : Gain  Gain=-1
  sliding friction coefficient : Gain  Gain=mu_slide
  tVec : Product  Inputs=*/  RndMeth=Zero
  v_n : DotProduct  OutDataTypeStr=Inherit: Inherit via internal rule
  v_nVec : Product  RndMeth=Zero
  v_tVec : Sum  Inputs=-+|
  RefPtFP [m m] : Outport  InitialOutput=[0 0]  VectorParamsAs1DForOutWhenUnconnected=off
      settings: AttributesFormatString=initial = '%<InitialOutput>'\nwhen disabled = '%<OutputWhenDisabled>'
  posFP [m m] : Outport  Port=2  InitialOutput=[0 0]  VectorParamsAs1DForOutWhenUnconnected=off
      settings: AttributesFormatString=initial = '%<InitialOutput>'\nwhen disabled = '%<OutputWhenDisabled>'
  nVec FP [m m] : Outport  Port=3  InitialOutput=0  VectorParamsAs1DForOutWhenUnconnected=off
      settings: AttributesFormatString=initial = '%<InitialOutput>'\nwhen disabled = '%<OutputWhenDisabled>'
  Stiction! : Outport  Port=4  OutputWhenDisabled=reset  InitialOutput=0  VectorParamsAs1DForOutWhenUnconnected=off
      settings: AttributesFormatString=initial = '%<InitialOutput>'\nwhen disabled = '%<OutputWhenDisabled>'
  F_t Slide [N N] : Outport  Port=5  OutputWhenDisabled=reset  InitialOutput=[0 0]  VectorParamsAs1DForOutWhenUnconnected=off
      settings: AttributesFormatString=initial = '%<InitialOutput>'\nwhen disabled = '%<OutputWhenDisabled>'
  F_n Slide [N N] : Outport  Port=6  OutputWhenDisabled=reset  InitialOutput=[0 0]  VectorParamsAs1DForOutWhenUnconnected=off
      settings: AttributesFormatString=initial = '%<InitialOutput>'\nwhen disabled = '%<OutputWhenDisabled>'
  wires:
  Normal Axis Ground Force/1 -> sliding friction coefficient/1, Product1/2
  Product/1 -> F_t Slide [N N]/1
  FixPt Relational Operator/1 -> Stiction!/1
  Memory/1 -> FixPt Relational Operator/2
  Negative/1 -> FixPt Relational Operator/1, Memory/1
  Vector Norm/1(norm) -> Sum/1, Switch/2, Mux2/2
  Sum/1 -> Negative/1
  Constant/1 -> Sum/2
  Mux1/1 -> Normal Axis Ground Force/1
  Gain3/1 -> Mux1/1
  Gain4/1 -> Mux1/2
  nVec [m m]/1 -> v_n/1, v_nVec/2, d_n/2, Product1/1, nVec FP [m m]/1
  d_n/1 -> Gain3/1
  vel [m/s m/s]/1 -> v_n/2, v_tVec/2
  v_n/1 -> Gain4/1, v_nVec/1
  v_nVec/1 -> v_tVec/1
  v_tVec/1 -> Vector Norm/1(vec), Mux2/1
  sliding friction coefficient/1 -> Product/1
  reverse direction/1 -> Product/2
  Product1/1 -> F_n Slide [N N]/1
  tVec/1 -> reverse direction/1
  Constant1/1 -> Switch/3
  Mux2/1 -> Switch/1
  Selector1/1 -> tVec/2
  Selector2/1 -> tVec/1
  pos [m m]/1 -> posFP [m m]/1, qnVec/1
  qnVec/1 -> d_n/1
  RefPt [m m]/1 -> qnVec/2, RefPtFP [m m]/1
  Switch/1 -> Selector2/1, Selector1/1
